simulink model "ecu_crankrd"  (R2026a)
settings: Solver=FixedStepDiscrete  StopTime=10  FixedStep=0.001  SampleTimeConstraint=STIndependent
Description:
  | Crank speed and angle from the decoder state. Source of truth for firmware/gen/ecu_crankrd.
settings Model: Creator=jj1001000  LastModifiedBy=jj1001000
settings OptimizationCC: DefaultUnderspecifiedDataType=single
settings DebuggingCC: ParameterPrecisionLossMsg=none
settings HardwareCC: ProdLargestAtomicInteger=Long  ProdLargestAtomicFloat=Double  ProdHWDeviceType=ARM Compatible->ARM Cortex-M
settings RTWCC: SystemTargetFile=ert.tlc  GenCodeOnly=on  Description=Embedded Coder
settings ERTTargetCC: UtilityFuncGeneration=Shared location  IncludeMdlTerminateFcn=off  CodeInterfacePackaging=Reusable function  SupportNonFinite=off

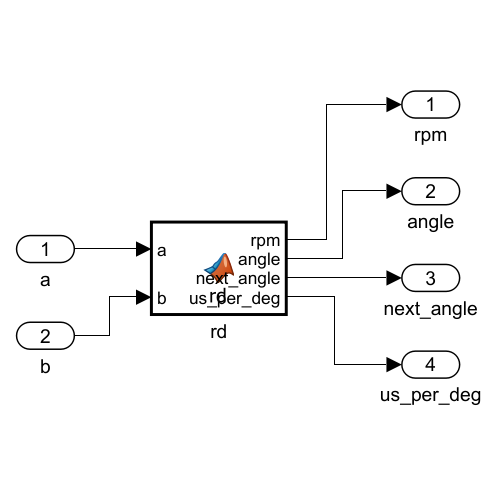
[thumbnail: Simulink's stored preview of the top-level diagram]
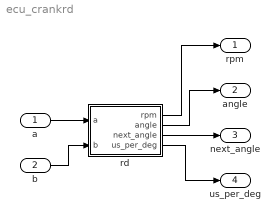
== system ecu_crankrd ==
  a : Inport  OutDataTypeStr=uint32  PortDimensions=8
  b : Inport  Port=2  OutDataTypeStr=uint8  PortDimensions=33
  rd : MATLAB Function  TreatAsAtomicUnit=on
  rpm : Outport  OutDataTypeStr=single
  angle : Outport  Port=2  OutDataTypeStr=single
  next_angle : Outport  Port=3  OutDataTypeStr=single
  us_per_deg : Outport  Port=4  OutDataTypeStr=single
  wires:
  b/1 -> rd/2(b)
  a/1 -> rd/1(a)
  rd/1(rpm) -> rpm/1
  rd/4(us_per_deg) -> us_per_deg/1
  rd/3(next_angle) -> next_angle/1
  rd/2(angle) -> angle/1

== matlab function ecu_crankrd/rd ==
  data: a input uint32; rpm output single; b input uint8; angle output single; next_angle output single; us_per_deg output single
function [rpm, angle, next_angle, us_per_deg] = rd(a, b)
%#codegen
WIN = int32(6); EDGES = uint8(58);
if b(7) < uint8(WIN)                    % nper
    rpm = single(0);
else
    us = uint32(0); deg = uint32(0);
    for i = int32(1):WIN
        us = us + a(2 + i); deg = deg + uint32(b(i));
    end
    rpm = single(deg) / single(us) * single(1e6) / single(6);
end
angle = single(b(14)) * single(360) + single(b(10)) * single(6);
if b(10) == EDGES - uint8(1)
    next_angle = angle + single(18);
else
    next_angle = angle + single(6);
end
if rpm > single(0)
    us_per_deg = single(1e6) / (rpm * single(6));
else
    us_per_deg = single(0);
end
